simulink model "simulation"  (R2025a)
settings: Solver=VariableStepAuto  StartTime=0.0  StopTime=60  RelTol=1e-3
values from neighbouring files (symbols this model uses):
  A_lat_SI = diag(1./lat_inputs)*A_lat_english*diag(outputs)    [main.m]
  A_lon_SI = diag(1./lon_inputs)*A_lon_english*diag(outputs)    [main.m]
  F_aero_trim = [ -D_trim * cos(alpha_trim) + L_trim * sin(alpha_trim) ... (first row only)    [main.m]
  g = 9.81    [main.m]
  mass = (weight_lbf/32.2)*slug_to_kg    (= 288524.180485)    [main.m]
  vel0 = [V_trim*cos(alpha_trim) 0 V_trim*sin(alpha_trim)]    [main.m]
libraries: aerolibanimutils x1
settings Model: Creator=darpansingh  LastModifiedBy=lilos

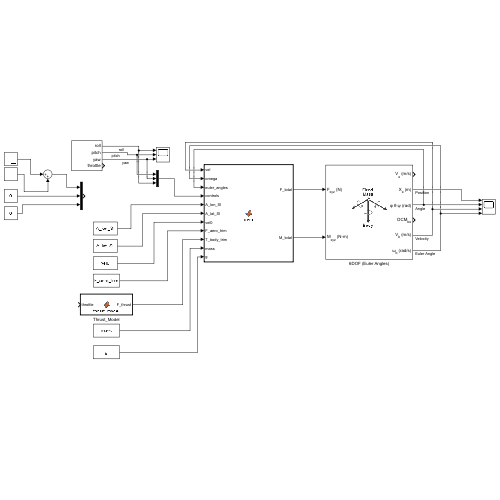
[thumbnail: Simulink's stored preview of the top-level diagram]
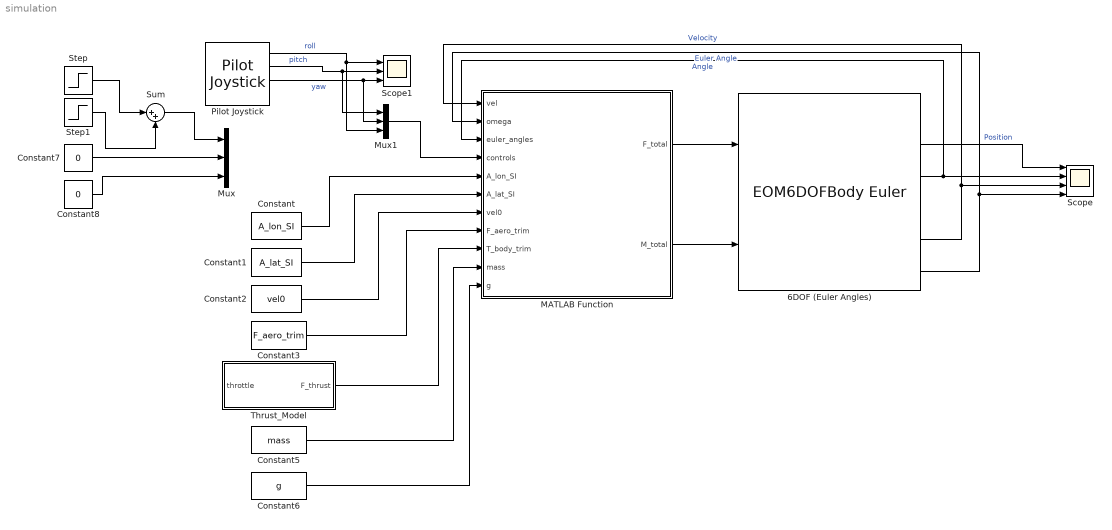
== system simulation ==
  6DOF (Euler Angles) : EOM6DOFBodyEuler  xme_0=pos0  Vm_0=vel0  eul_0=euler0  pm_0=omega0  mass_0=mass  inertia=inertia
  Constant : Constant  Value=A_lon_SI
  Constant1 : Constant  Value=A_lat_SI
  Constant2 : Constant  Value=vel0
  Constant3 : Constant  Value=F_aero_trim
  Constant5 : Constant  Value=mass
  Constant6 : Constant  Value=g
  Constant7 : Constant  Value=0
  Constant8 : Constant  Value=0
  MATLAB Function : MATLAB Function  TreatAsAtomicUnit=on
  Mux : Mux  Inputs=3
  Mux1 : Mux  Inputs=3
  Pilot Joystick : aerolibanimutils/Pilot Joystick  JoystickID=Joystick1  OutputConfiguration=FourAxis  SampleTime=1/30
  Scope : Scope  NumInputPorts=4
      settings: ActiveDisplayYMinimum=-7425.2719364521672  ActiveDisplayYMaximum=5867.4474280695022
  Scope1 : Scope  NumInputPorts=3
      settings: ActiveDisplayYMinimum=-1.25  ActiveDisplayYMaximum=1.25
  Step : Step  Time=5  After=-deg2rad(1)  SampleTime=0
  Step1 : Step  Time=6  After=deg2rad(1)  SampleTime=0
  Sum : Sum  Inputs=|++
  Thrust_Model : MATLAB Function  TreatAsAtomicUnit=on
  wires:
  MATLAB Function/1(F_total) -> 6DOF (Euler Angles)/1
  MATLAB Function/2(M_total) -> 6DOF (Euler Angles)/2
  6DOF (Euler Angles)/5 -> Scope/3, MATLAB Function/1(vel)  "Velocity"
  6DOF (Euler Angles)/6 -> Scope/4, MATLAB Function/2(omega)  "Euler Angle"
  6DOF (Euler Angles)/3 -> Scope/2, MATLAB Function/3(euler_angles)  "Angle"
  Constant/1 -> MATLAB Function/5(A_lon_SI)
  Constant1/1 -> MATLAB Function/6(A_lat_SI)
  Constant2/1 -> MATLAB Function/7(vel0)
  Constant3/1 -> MATLAB Function/8(F_aero_trim)
  Constant5/1 -> MATLAB Function/10(mass)
  Constant6/1 -> MATLAB Function/11(g)
  6DOF (Euler Angles)/2 -> Scope/1  "Position"
  Step/1 -> Sum/1
  Step1/1 -> Sum/2
  Sum/1 -> Mux/1
  Constant7/1 -> Mux/2
  Constant8/1 -> Mux/3
  Pilot Joystick/1 -> Mux1/3, Scope1/1  "roll"
  Pilot Joystick/2 -> Mux1/1, Scope1/2  "pitch"
  Pilot Joystick/3 -> Mux1/2, Scope1/3  "yaw"
  Thrust_Model/1(F_thrust) -> MATLAB Function/9(T_body_trim)
  Mux1/1 -> MATLAB Function/4(controls)

== matlab function simulation/MATLAB Function ==
  data: vel input; F_total output; omega input; euler_angles input; controls input; A_lon_SI input; A_lat_SI input; vel0 input; F_aero_trim input; T_body_trim input; mass input; g input; M_total output
function [F_total, M_total] = aero(vel, omega, euler_angles, controls, ...
    A_lon_SI, A_lat_SI, vel0, F_aero_trim, T_body_trim, mass, g)

% Call aero.m (the loop model script)
[F_total, M_total] = aero( ...
    vel, omega, euler_angles, controls, ...
    A_lon_SI, A_lat_SI, vel0, ...
    F_aero_trim, T_body_trim, mass, g);

end

== matlab function simulation/Thrust_Model ==
  data: throttle input; F_thrust output size=3; T_max parameter
function F_thrust = thrust_model(throttle, T_max)
%#codegen
% Placeholder propulsion model: 4x P&W JT9D-3, LINEAR throttle law.
%   throttle : 0..1 command from the Throttle block (0 = idle, 1 = max)
%   T_max    : total max thrust at the trim condition [N] (parameter, set in main.m)
%   F_thrust : body-axis thrust force [N], along +x_b through the CG
% Replace the linear law with the JT9D throttle curve later.

th = min(max(throttle, 0), 1);   % clip to the physical lever range
F_thrust = [th*T_max; 0; 0];
end
